simulink model "Robot_Control"  (R2026a)
settings: Solver=FixedStepDiscrete  StopTime=inf  FixedStep=t_sample
undefined symbols (not defined in the file): t_sample
settings Model: Creator=FIRSTMentor  LastModifiedBy=ander
settings OptimizationCC: StrengthReduction=on  OptimizationPriority=Speed  MultiThreadedLoops=on  AutoScheduleForLoops=on  UseRestrictQualifier=on
settings HardwareCC: ProdLargestAtomicInteger=Long  ProdHWDeviceType=ARM Compatible->ARM 7
settings RTWCC: SystemTargetFile=ert.tlc  GenCodeOnly=on  Toolchain=MinGW64 | gmake (64-bit Windows)  Description=Embedded Coder
settings ERTTargetCC: DynamicArrayContainerType=coder::array  UtilityFuncGeneration=Shared location  SupportVariableSizeSignals=on  ParenthesesLevel=Maximum
settings SimscapeCC: SimscapeNominalValues="[{\"value\":\"1\",\"unit\":\"A\"},{\"value\":\"1\",\"unit\":\"bar\"},{\"value\":\"1\",\"unit\":\"cm^2\"},{\"value\":\"1\",\"unit\":\"cm^3/s\"},{\"value\":\"1\",\"unit\":\"kJ/kg\"},{\"value\":\"1\",\"unit\":\"kW\"},{\"value\":\"1\",\"unit\":\"l\"},{\"value\":\"1\",\"unit\":\"N\"},{\"value\":\"1\",\"unit\":\"N*m\"},{\"value\":\"1\",\"unit\":\"V\"}]"  SimscapeLogType=none  SimscapeLogDataHistory=5000.0

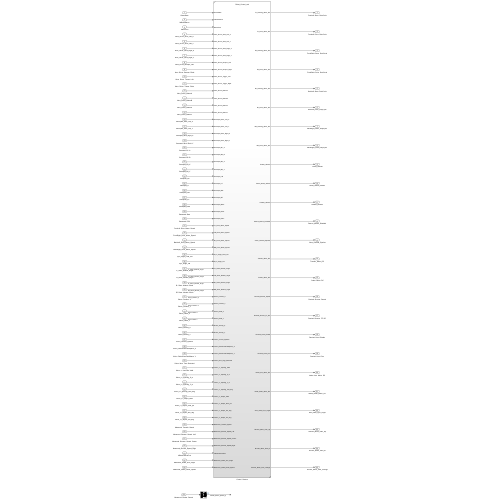
[thumbnail: Simulink's stored preview of the top-level diagram]
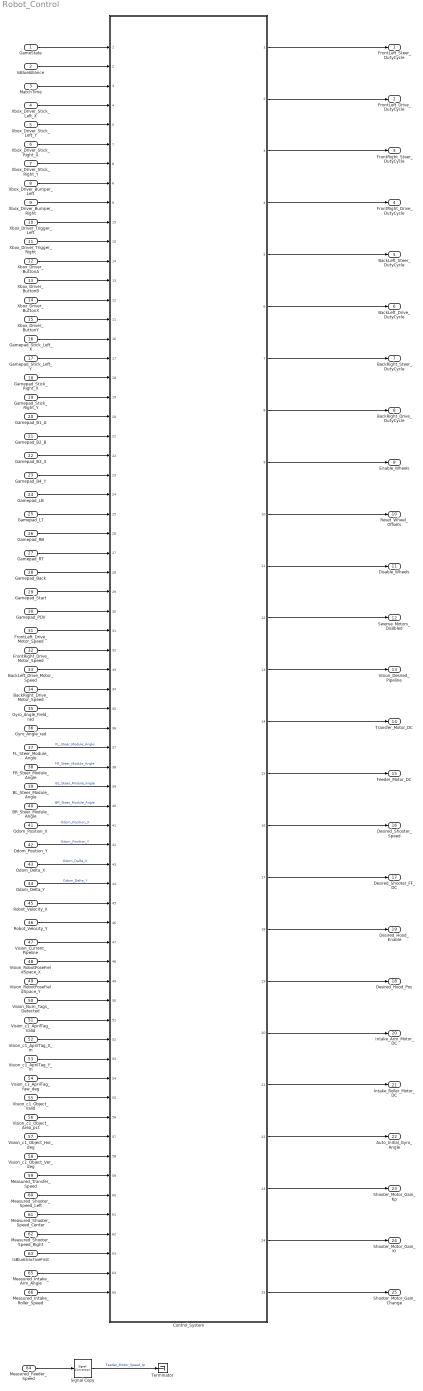
== system Robot_Control ==
  GameState : Inport
  IsBlueAlliance : Inport  Port=2
  MatchTime : Inport  Port=3
  Xbox_Driver_Stick_Left_X : Inport  Port=4
  Xbox_Driver_Stick_Left_Y : Inport  Port=5
  Xbox_Driver_Stick_Right_X : Inport  Port=6
  Xbox_Driver_Stick_Right_Y : Inport  Port=7
  Xbox_Driver_Bumper_Left : Inport  Port=8
  Xbox_Driver_Bumper_Right : Inport  Port=9
  Xbox_Driver_Trigger_Left : Inport  Port=10
  Xbox_Driver_Trigger_Right : Inport  Port=11
  Xbox_Driver_ButtonA : Inport  Port=12
  Xbox_Driver_ButtonB : Inport  Port=13
  Xbox_Driver_ButtonX : Inport  Port=14
  Xbox_Driver_ButtonY : Inport  Port=15
  Gamepad_Stick_Left_X : Inport  Port=16
  Gamepad_Stick_Left_Y : Inport  Port=17
  Gamepad_Stick_Right_X : Inport  Port=18
  Gamepad_Stick_Right_Y : Inport  Port=19
  Gamepad_B1_A : Inport  Port=20
  Gamepad_B2_B : Inport  Port=21
  Gamepad_B3_X : Inport  Port=22
  Gamepad_B4_Y : Inport  Port=23
  Gamepad_LB : Inport  Port=24
  Gamepad_LT : Inport  Port=25
  Gamepad_RB : Inport  Port=26
  Gamepad_RT : Inport  Port=27
  Gamepad_Back : Inport  Port=28
  Gamepad_Start : Inport  Port=29
  Gamepad_POV : Inport  Port=30
  FrontLeft_Drive_Motor_Speed : Inport  Port=31
  FrontRight_Drive_Motor_Speed : Inport  Port=32
  BackLeft_Drive_Motor_Speed : Inport  Port=33
  BackRight_Drive_Motor_Speed : Inport  Port=34
  Gyro_Angle_Field_rad : Inport  Port=35
  Gyro_Angle_rad : Inport  Port=36
  FL_Steer_Module_Angle : Inport  Port=37
  FR_Steer_Module_Angle : Inport  Port=38
  BL_Steer_Module_Angle : Inport  Port=39
  BR_Steer_Module_Angle : Inport  Port=40
  Odom_Position_X : Inport  Port=41
  Odom_Position_Y : Inport  Port=42
  Odom_Delta_X : Inport  Port=43
  Odom_Delta_Y : Inport  Port=44
  Robot_Velocity_X : Inport  Port=45
  Robot_Velocity_Y : Inport  Port=46
  Vision_Current_Pipeline : Inport  Port=47
  Vision_RobotPoseFieldSpace_X : Inport  Port=48
  Vision_RobotPoseFieldSpace_Y : Inport  Port=49
  Vision_Num_Tags_Detected : Inport  Port=50
  Vision_c1_AprilTag_Valid : Inport  Port=51
  Vision_c1_AprilTag_X_m : Inport  Port=52
  Vision_c1_AprilTag_Y_m : Inport  Port=53
  Vision_c1_AprilTag_Yaw_deg : Inport  Port=54
  Vision_c1_Object_Valid : Inport  Port=55
  Vision_c1_Object_Area_pct : Inport  Port=56
  Vision_c1_Object_Hor_deg : Inport  Port=57
  Vision_c1_Object_Ver_deg : Inport  Port=58
  Measured_Transfer_Speed : Inport  Port=59
  Measured_Shooter_Speed_Left : Inport  Port=60
  Measured_Shooter_Speed_Center : Inport  Port=61
  Measured_Shooter_Speed_Right : Inport  Port=62
  IsBlueInactiveFirst : Inport  Port=63
  Measured_Feeder_Speed : Inport  Port=64
  Measured_Intake_Arm_Angle : Inport  Port=65
  Measured_Intake_Roller_Speed : Inport  Port=66
  Control_System : Subsystem  SystemSampleTime=t_sample  RTWFcnName=Model_Step  ReferencedSubsystem=Robot_Control_sub
      settings: RTWSystemCode=Nonreusable function  RTWFcnNameOpts=User specified  PortSchema="{\"entries\":[{\"content\":{\"sides\":[{\"content\":{\"connectorIds\":[\"In1\",\"In2\",\"In3\",\"In4\",\"In5\",\"In7\",\"In8\",\"In6\",\"In9\",\"In15\",\"In10\",\"In14\",\"In13\",\"In12\",\"In11\",\"In16\",\"In17\",\"In18\",\"In19\",\"In20\",\"In21\",\"In22\",\"In23\",\"In24\",\"In25\",\"In26\",\"In27\",\"In28\",\"In29\",\"In30\",\"In31\",\"In32\",\"In33\",\"In34\",\"In35\",\"In36\",\"In37\",\"In38\",\"In39\",\"In40\",\"In41\",\"In42\",\"In43\",\"In44\",\"In45\",\"In46\",\"In47\",\"In48\",\"In49\",\"In50\",\"In51\",\"In52\",\"In53\",\"In54\",\"In55\",\"In56\",\"In57\",\"In58\",\"In59\",\"In60\",\"In61\",\"In62\",\"In63\",\"In64\",\"In65\"]},\"type\":\"ConnectorPlacement.EquallySpacedRectSide\",\"uuid\":\"0ce51be8-83c2-42fc-954e-b076ec44321c\"},{\"content\":{\"connectorIds\":[\"Out1\",\"Out2\",\"Out3\",\"Out4\",\"Out5\",\"Out6\",\"Out7\",\"Out8\",\"Out9\",\"Out10\",\"Out11\",\"Out12\",\"Out13\",\"Out14\",\"Out15\",\"Out16\",\"Out17\",\"Out18\",\"Out19\",\"Out20\",\"Out21\",\"Out22\",\"Out23\",\"Out24\",\"Out25\"],\"side\":\"RIGHT\"},\"type\":\"ConnectorPlacement.EquallySpacedRectSide\",\"uuid\":\"0407e9e6-8138-44a9-ba00-a0786243f02f\"},{\"content\":{\"side\":\"TOP\"},\"type\":\"ConnectorPlacement.EquallySpacedRectSide\",\"uuid\":\"df4351c2-d9a6-4781-982d-df788ecced56\"}]},\"type\":\"ConnectorPlacement.EquallySpacedConnector\",\"uuid\":\"1484ae1b-922e-4e19-81fe-de52dd6e0552\"}],\"packageUris\":[\"http://schema.mathworks.com/mf0/Connector/R2020b\"],\"version\":\"1.0\"}"
  Signal Copy : SignalConversion  OverrideOpt=off
  Terminator : Terminator
  FrontLeft_Steer_DutyCycle : Outport
  FrontLeft_Drive_DutyCycle : Outport  Port=2
  FrontRight_Steer_DutyCycle : Outport  Port=3
  FrontRight_Drive_DutyCycle : Outport  Port=4
  BackLeft_Steer_DutyCycle : Outport  Port=5
  BackLeft_Drive_DutyCycle : Outport  Port=6
  BackRight_Steer_DutyCycle : Outport  Port=7
  BackRight_Drive_DutyCycle : Outport  Port=8
  Enable_Wheels : Outport  Port=9
  Reset_Wheel_Offsets : Outport  Port=10
  Disable_Wheels : Outport  Port=11
  Swerve_Motors_Disabled : Outport  Port=12
  Vision_Desired_Pipeline : Outport  Port=13
  Transfer_Motor_DC : Outport  Port=14
  Feeder_Motor_DC : Outport  Port=15
  Desired_Shooter_Speed : Outport  Port=16
  Desired_Shooter_FF_DC : Outport  Port=17
  Desired_Hood_Pos : Outport  Port=18
  Desired_Hood_Enable : Outport  Port=19
  Intake_Arm_Motor_DC : Outport  Port=20
  Intake_Roller_Motor_DC : Outport  Port=21
  Auto_Initial_Gyro_Angle : Outport  Port=22
  Shooter_Motor_Gain_Kp : Outport  Port=23
  Shooter_Motor_Gain_Ki : Outport  Port=24
  Shooter_Motor_Gain_Change : Outport  Port=25
  wires:
  Odom_Delta_Y/1 -> Control_System/44  "Odom_Delta_Y"
  Xbox_Driver_Trigger_Right/1 -> Control_System/10
  Xbox_Driver_Stick_Right_Y/1 -> Control_System/8
  Xbox_Driver_ButtonX/1 -> Control_System/12
  Xbox_Driver_Stick_Left_Y/1 -> Control_System/5
  Xbox_Driver_Stick_Left_X/1 -> Control_System/4
  Xbox_Driver_Trigger_Left/1 -> Control_System/15
  FrontRight_Drive_Motor_Speed/1 -> Control_System/32
  MatchTime/1 -> Control_System/3
  Xbox_Driver_ButtonA/1 -> Control_System/14
  Control_System/6 -> BackLeft_Drive_DutyCycle/1
  Control_System/9 -> Enable_Wheels/1
  FrontLeft_Drive_Motor_Speed/1 -> Control_System/31
  Gamepad_POV/1 -> Control_System/30
  Vision_Num_Tags_Detected/1 -> Control_System/50
  Vision_c1_AprilTag_Y_m/1 -> Control_System/53
  Vision_Current_Pipeline/1 -> Control_System/47
  Gyro_Angle_Field_rad/1 -> Control_System/35
  Vision_c1_AprilTag_X_m/1 -> Control_System/52
  Gamepad_Stick_Right_X/1 -> Control_System/18
  Gamepad_Start/1 -> Control_System/29
  Control_System/10 -> Reset_Wheel_Offsets/1
  Gamepad_B2_B/1 -> Control_System/21
  Gamepad_RB/1 -> Control_System/26
  Control_System/1 -> FrontLeft_Steer_DutyCycle/1
  Control_System/4 -> FrontRight_Drive_DutyCycle/1
  IsBlueAlliance/1 -> Control_System/2
  Gamepad_RT/1 -> Control_System/27
  Control_System/5 -> BackLeft_Steer_DutyCycle/1
  Control_System/13 -> Vision_Desired_Pipeline/1
  Control_System/11 -> Disable_Wheels/1
  Control_System/7 -> BackRight_Steer_DutyCycle/1
  Xbox_Driver_ButtonB/1 -> Control_System/13
  Control_System/2 -> FrontLeft_Drive_DutyCycle/1
  BackRight_Drive_Motor_Speed/1 -> Control_System/34
  Gamepad_Stick_Right_Y/1 -> Control_System/19
  Gamepad_B4_Y/1 -> Control_System/23
  Gamepad_B1_A/1 -> Control_System/20
  Vision_RobotPoseFieldSpace_Y/1 -> Control_System/49
  BackLeft_Drive_Motor_Speed/1 -> Control_System/33
  Gamepad_LT/1 -> Control_System/25
  Vision_RobotPoseFieldSpace_X/1 -> Control_System/48
  Gamepad_B3_X/1 -> Control_System/22
  Control_System/3 -> FrontRight_Steer_DutyCycle/1
  Control_System/12 -> Swerve_Motors_Disabled/1
  GameState/1 -> Control_System/1
  FL_Steer_Module_Angle/1 -> Control_System/37  "FL_Steer_Module_Angle"
  Odom_Delta_X/1 -> Control_System/43  "Odom_Delta_X"
  Gamepad_Stick_Left_Y/1 -> Control_System/17
  Gamepad_LB/1 -> Control_System/24
  Xbox_Driver_ButtonY/1 -> Control_System/11
  Gyro_Angle_rad/1 -> Control_System/36
  Odom_Position_Y/1 -> Control_System/42  "Odom_Position_Y"
  Odom_Position_X/1 -> Control_System/41  "Odom_Position_X"
  BR_Steer_Module_Angle/1 -> Control_System/40  "BR_Steer_Module_Angle"
  Gamepad_Stick_Left_X/1 -> Control_System/16
  BL_Steer_Module_Angle/1 -> Control_System/39  "BL_Steer_Module_Angle"
  Control_System/8 -> BackRight_Drive_DutyCycle/1
  Gamepad_Back/1 -> Control_System/28
  FR_Steer_Module_Angle/1 -> Control_System/38  "FR_Steer_Module_Angle"
  Xbox_Driver_Stick_Right_X/1 -> Control_System/7
  Vision_c1_AprilTag_Yaw_deg/1 -> Control_System/54
  Vision_c1_Object_Area_pct/1 -> Control_System/56
  Vision_c1_Object_Hor_deg/1 -> Control_System/57
  Vision_c1_Object_Ver_deg/1 -> Control_System/58
  Vision_c1_AprilTag_Valid/1 -> Control_System/51
  Vision_c1_Object_Valid/1 -> Control_System/55
  Measured_Transfer_Speed/1 -> Control_System/59
  Measured_Shooter_Speed_Left/1 -> Control_System/60
  Measured_Shooter_Speed_Center/1 -> Control_System/61
  Measured_Shooter_Speed_Right/1 -> Control_System/62
  Robot_Velocity_X/1 -> Control_System/45
  Robot_Velocity_Y/1 -> Control_System/46
  Measured_Feeder_Speed/1 -> Signal Copy/1
  Signal Copy/1 -> Terminator/1  "Feeder_Motor_Speed_tp"
  Control_System/19 -> Desired_Hood_Pos/1
  Control_System/14 -> Transfer_Motor_DC/1
  Control_System/15 -> Feeder_Motor_DC/1
  Control_System/16 -> Desired_Shooter_Speed/1
  Control_System/17 -> Desired_Shooter_FF_DC/1
  Control_System/18 -> Desired_Hood_Enable/1
  IsBlueInactiveFirst/1 -> Control_System/63
  Measured_Intake_Roller_Speed/1 -> Control_System/65
  Measured_Intake_Arm_Angle/1 -> Control_System/64
  Control_System/21 -> Intake_Roller_Motor_DC/1
  Control_System/20 -> Intake_Arm_Motor_DC/1
  Control_System/22 -> Auto_Initial_Gyro_Angle/1
  Control_System/25 -> Shooter_Motor_Gain_Change/1
  Control_System/23 -> Shooter_Motor_Gain_Kp/1
  Control_System/24 -> Shooter_Motor_Gain_Ki/1
  Xbox_Driver_Bumper_Left/1 -> Control_System/6
  Xbox_Driver_Bumper_Right/1 -> Control_System/9
